simulink model "untitled1"  (R2023b)
settings: Solver=VariableStepAuto  StartTime=0.0  StopTime=10.0  RelTol=1e-3
settings Model: Creator=12427  LastModifiedBy=12427

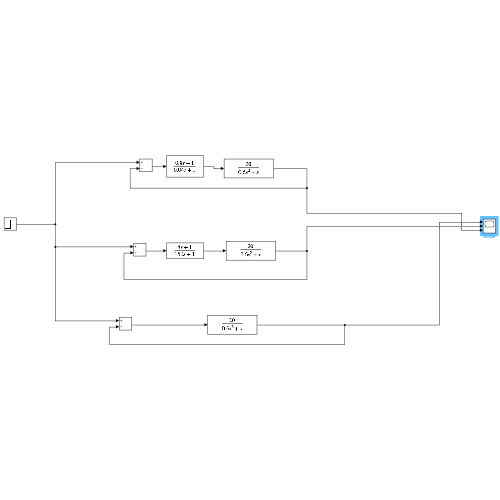
[thumbnail: Simulink's stored preview of the top-level diagram]
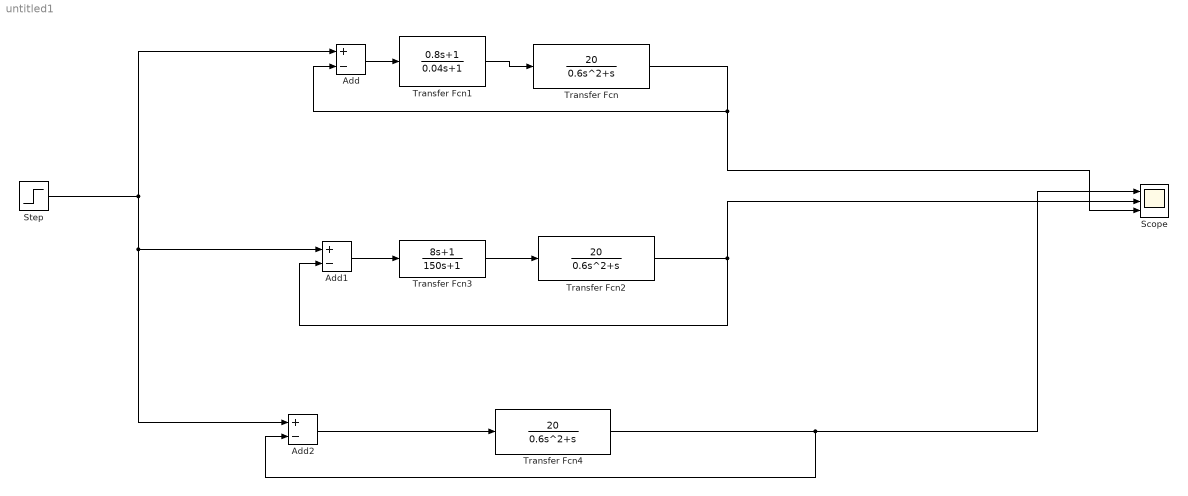
== system untitled1 ==
  Add : Sum  Inputs=+-
  Add1 : Sum  Inputs=+-
  Add2 : Sum  Inputs=+-
  Scope : Scope  NumInputPorts=3
  Step : Step  Time=0  SampleTime=0.001
  Transfer Fcn : TransferFcn  Numerator=[20]  Denominator=[0.6 1 0]
  Transfer Fcn1 : TransferFcn  Numerator=[0.8 1]  Denominator=[0.04 1]
  Transfer Fcn2 : TransferFcn  Numerator=[20]  Denominator=[0.6 1 0]
  Transfer Fcn3 : TransferFcn  Numerator=[8 1]  Denominator=[150 1]
  Transfer Fcn4 : TransferFcn  Numerator=[20]  Denominator=[0.6 1 0]
  wires:
  Add2/1 -> Transfer Fcn4/1
  Transfer Fcn4/1 -> Add2/2, Scope/1
  Transfer Fcn/1 -> Add/2, Scope/3
  Transfer Fcn1/1 -> Transfer Fcn/1
  Add/1 -> Transfer Fcn1/1
  Step/1 -> Add/1, Add1/1, Add2/1
  Transfer Fcn2/1 -> Add1/2, Scope/2
  Add1/1 -> Transfer Fcn3/1
  Transfer Fcn3/1 -> Transfer Fcn2/1
